simulink library "lib_Grid_DC_Dynamic"  (R2026a)
settings: Solver=VariableStepAuto
undefined symbols (not defined in the file): DC, From_nodes, Load_busesDC, op_Grid_DC_Dynamic, R_Loads_DC
settings Model: Creator=atomas  LastModifiedBy=atomas

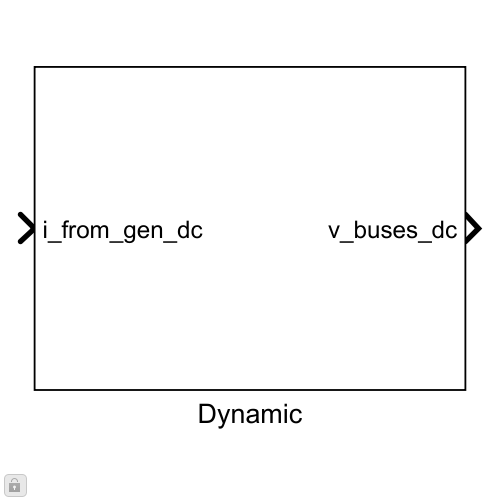
[thumbnail: Simulink's stored preview of the top-level diagram]
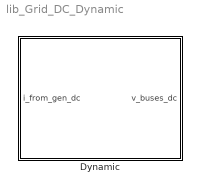
== system lib_Grid_DC_Dynamic ==
  Dynamic : Subsystem  VariantControl=Dynamic

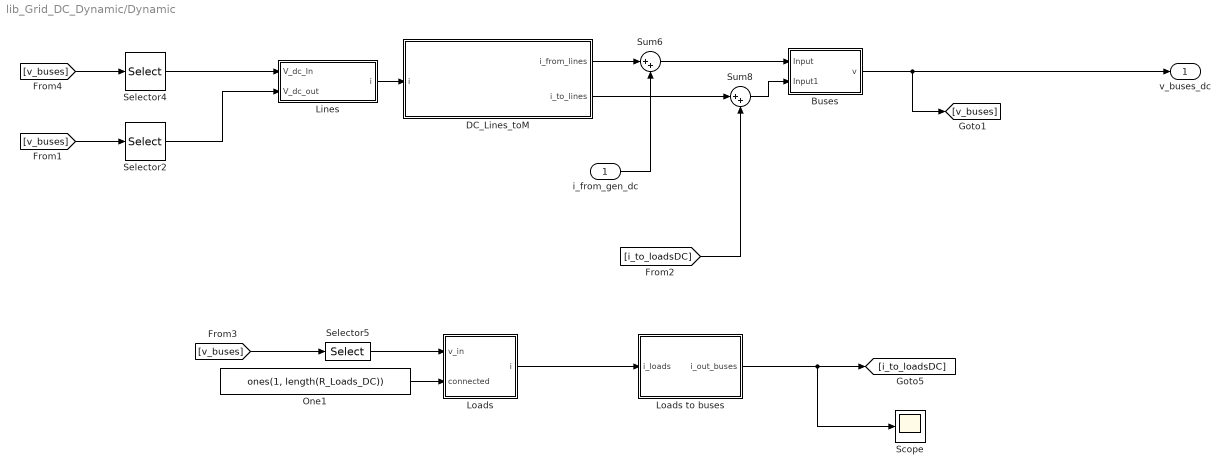
== system lib_Grid_DC_Dynamic/Dynamic ==
  i_from_gen_dc : Inport
  Buses : Subsystem
  DC_Lines_toM : Subsystem  TreatAsAtomicUnit=on
  Lines : Subsystem
  Loads : Subsystem
  Loads to buses : Subsystem
  One1 : Constant  Value=ones(1, length(R_Loads_DC))  VectorParams1D=off  OutDataTypeStr=Inherit: Inherit via back propagation
  Scope : Scope
      settings: ActiveDisplayYMinimum=-0.01246  ActiveDisplayYMaximum=0.11218
  Selector2 : Selector  NumberOfDimensions=2  InputPortWidth=Nnodes  IndexOptions=Select all,Index vector (dialog)  Indices=From_nodes,DC.to  OutputSizes=1,1
  Selector4 : Selector  NumberOfDimensions=2  InputPortWidth=Nnodes  IndexOptions=Select all,Index vector (dialog)  Indices=From_nodes,DC.from  OutputSizes=1,1
  Selector5 : Selector  NumberOfDimensions=2  InputPortWidth=Nnodes  IndexOptions=Select all,Index vector (dialog)  Indices=1,Load_busesDC  OutputSizes=1,1
  Sum6 : Sum  Inputs=|++
  Sum8 : Sum  Inputs=|++
  v_buses_dc : Outport
  wires:
  Buses/1(v) -> v_buses_dc/1, [v_buses]
  [v_buses] -> Selector2/1
  Selector2/1 -> Lines/2(V_dc_out)
  Sum6/1 -> Buses/1(Input)
  Selector4/1 -> Lines/1(V_dc_In)
  Loads/1(i) -> Loads to buses/1(i_loads)
  Selector5/1 -> Loads/1(v_in)
  i_from_gen_dc/1 -> Sum6/2
  Sum8/1 -> Buses/2(Input1)
  DC_Lines_toM/2(i_to_lines) -> Sum8/1
  DC_Lines_toM/1(i_from_lines) -> Sum6/1
  [v_buses] -> Selector4/1
  [i_to_loadsDC] -> Sum8/2
  Lines/1(i) -> DC_Lines_toM/1(i)
  One1/1 -> Loads/2(connected)
  Loads to buses/1(i_out_buses) -> Scope/1, [i_to_loadsDC]
  [v_buses] -> Selector5/1

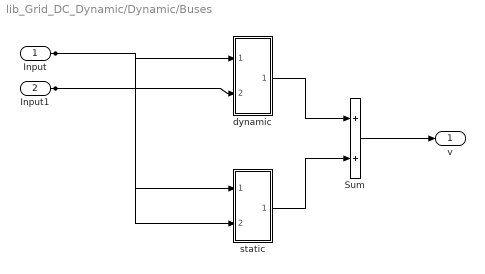
== system lib_Grid_DC_Dynamic/Dynamic/Buses ==
  Input : Inport
  Input1 : Inport  Port=2
  Sum : Sum
  dynamic : Subsystem  Variant=on
  static : Subsystem  Variant=on
  v : Outport
  wires:
  static/1(Out1) -> Sum/2
  Input1/1 -> static/2(In2), dynamic/2(In2)
  Input/1 -> static/1(In1), dynamic/1(In1)
  dynamic/1(Out1) -> Sum/1
  Sum/1 -> v/1

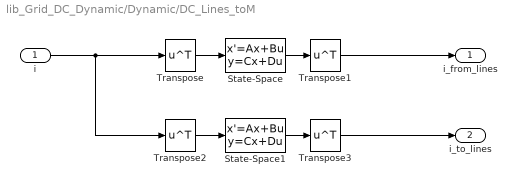
== system lib_Grid_DC_Dynamic/Dynamic/DC_Lines_toM ==
  i : Inport
  State-Space : StateSpace  A=[]  B=[]  C=[]  D=DC.Lines_toM  InitialCondition=0  ParameterTunability=Optimized
  State-Space1 : StateSpace  A=[]  B=[]  C=[]  D=DC.Lines_fromM  InitialCondition=0  ParameterTunability=Optimized
  Transpose{,1..3} (4 alike) : Math  Operator=transpose
  i_from_lines : Outport
  i_to_lines : Outport  Port=2
  wires:
  Transpose2/1 -> State-Space1/1
  i/1 -> Transpose2/1, Transpose/1
  Transpose3/1 -> i_to_lines/1
  Transpose/1 -> State-Space/1
  State-Space1/1 -> Transpose3/1
  State-Space/1 -> Transpose1/1
  Transpose1/1 -> i_from_lines/1

== system lib_Grid_DC_Dynamic/Dynamic/Lines ==
  V_dc_In : Inport
  V_dc_out : Inport  Port=2
  Dynamic : Subsystem  Variant=on
  Static : Subsystem  Variant=on
  Sum4 : Sum
  i : Outport
  wires:
  Static/1(Out1) -> Sum4/2
  V_dc_out/1 -> Static/2(In2), Dynamic/2(In2)
  V_dc_In/1 -> Static/1(In1), Dynamic/1(In1)
  Dynamic/1(Out1) -> Sum4/1
  Sum4/1 -> i/1

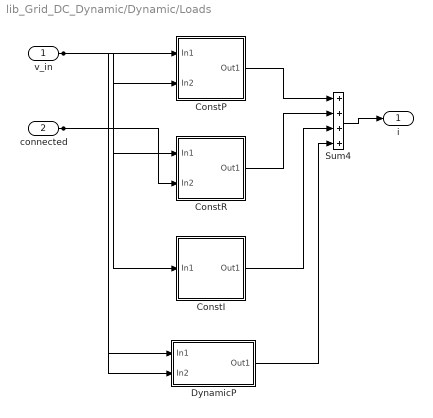
== system lib_Grid_DC_Dynamic/Dynamic/Loads ==
  v_in : Inport
  connected : Inport  Port=2
  ConstI : Subsystem  Variant=on
  ConstP : Subsystem  Variant=on
  ConstR : Subsystem  Variant=on
  DynamicP : Subsystem  Variant=on
  Sum4 : Sum  Inputs=++++
  i : Outport
  wires:
  DynamicP/1(Out1) -> Sum4/4
  connected/1 -> DynamicP/2(In2), ConstI/1(In1), ConstP/2(In2), ConstR/2(In2)
  v_in/1 -> DynamicP/1(In1), ConstP/1(In1), ConstR/1(In1)
  ConstI/1(Out1) -> Sum4/3
  ConstP/1(Out1) -> Sum4/1
  ConstR/1(Out1) -> Sum4/2
  Sum4/1 -> i/1

== system lib_Grid_DC_Dynamic/Dynamic/Loads to buses ==
  i_loads : Inport
  LoadsM : Subsystem  TreatAsAtomicUnit=on
  i_out_buses : Outport
  wires:
  i_loads/1 -> LoadsM/1(i)
  LoadsM/1(i_out_buses) -> i_out_buses/1

== system lib_Grid_DC_Dynamic/Dynamic/Buses/dynamic ==
  note: 1) Add Subsystem or Model blocks as valid variant choices.
      | 2) You cannot connect blocks at this level. At simulation, connectivity is automatically
      | determined, based on the active variant and port name matching.
  In1 : Inport
  In2 : Inport  Port=2
  Active : Subsystem  VariantControl=has_busDC_c1 == 1
  Bypass : Subsystem  VariantControl=(default)
  Out1 : Outport

== system lib_Grid_DC_Dynamic/Dynamic/Buses/static ==
  note: 1) Add Subsystem or Model blocks as valid variant choices.
      | 2) You cannot connect blocks at this level. At simulation, connectivity is automatically
      | determined, based on the active variant and port name matching.
  In1 : Inport
  In2 : Inport  Port=2
  Active : Subsystem  VariantControl=has_busDC_c2 == 1
  Bypass : Subsystem  VariantControl=(default)
  Out1 : Outport

== system lib_Grid_DC_Dynamic/Dynamic/Lines/Dynamic ==
  note: 1) Add Subsystem or Model blocks as valid variant choices.
      | 2) You cannot connect blocks at this level. At simulation, connectivity is automatically
      | determined, based on the active variant and port name matching.
  In1 : Inport
  In2 : Inport  Port=2
  Active : Subsystem  VariantControl=has_lineDC_c1 == 1
  Bypass : Subsystem  VariantControl=(default)
  Out1 : Outport

== system lib_Grid_DC_Dynamic/Dynamic/Lines/Static ==
  note: 1) Add Subsystem or Model blocks as valid variant choices.
      | 2) You cannot connect blocks at this level. At simulation, connectivity is automatically
      | determined, based on the active variant and port name matching.
  In1 : Inport
  In2 : Inport  Port=2
  Active : Subsystem  VariantControl=has_lineDC_c2 == 1
  Bypass : Subsystem  VariantControl=(default)
  Out1 : Outport

== system lib_Grid_DC_Dynamic/Dynamic/Loads/ConstI ==
  note: 1) Add Subsystem or Model blocks as valid variant choices.
      | 2) You cannot connect blocks at this level. At simulation, connectivity is automatically
      | determined, based on the active variant and port name matching.
  In1 : Inport
  Active : Subsystem  VariantControl=has_loadDC_c3 == 1
  Bypass : Subsystem  VariantControl=(default)
  Out1 : Outport

== system lib_Grid_DC_Dynamic/Dynamic/Loads/ConstP ==
  note: 1) Add Subsystem or Model blocks as valid variant choices.
      | 2) You cannot connect blocks at this level. At simulation, connectivity is automatically
      | determined, based on the active variant and port name matching.
  In1 : Inport
  In2 : Inport  Port=2
  Active : Subsystem  VariantControl=has_loadDC_c2 == 1
  Bypass : Subsystem  VariantControl=(default)
  Out1 : Outport

== system lib_Grid_DC_Dynamic/Dynamic/Loads/ConstR ==
  note: 1) Add Subsystem or Model blocks as valid variant choices.
      | 2) You cannot connect blocks at this level. At simulation, connectivity is automatically
      | determined, based on the active variant and port name matching.
  In1 : Inport
  In2 : Inport  Port=2
  Active : Subsystem  VariantControl=has_loadDC_c1 == 1
  Bypass : Subsystem  VariantControl=(default)
  Out1 : Outport

== system lib_Grid_DC_Dynamic/Dynamic/Loads/DynamicP ==
  note: 1) Add Subsystem or Model blocks as valid variant choices.
      | 2) You cannot connect blocks at this level. At simulation, connectivity is automatically
      | determined, based on the active variant and port name matching.
  In1 : Inport
  In2 : Inport  Port=2
  Active : Subsystem  VariantControl=has_loadDC_c4 == 1
  Bypass : Subsystem  VariantControl=(default)
  Out1 : Outport

== system lib_Grid_DC_Dynamic/Dynamic/Loads to buses/LoadsM ==
  i : Inport  Partition=on  PartitionDimension=1  PartitionWidth=1  PartitionOffset=0
  Assignment : Assignment  DiagnosticForDimensions=Warning  IndexOptions=Index vector (dialog)  Indices=Load_busesDC  OutputSizes=1
  For Each : ForEach  DisableCoverage=on
  Zero : Constant  Value=zeros(1,DC.Nbuses)  VectorParams1D=off  OutDataTypeStr=Inherit: Inherit via back propagation
  i_out_buses : Outport  ConcatenationDimension=1
  wires:
  Assignment/1 -> i_out_buses/1
  i/1 -> Assignment/2
  Zero/1 -> Assignment/1

== system lib_Grid_DC_Dynamic/Dynamic/Buses/dynamic/Active ==
  In1 : Inport
  In2 : Inport  Port=2
  Impl : Subsystem
  Out1 : Outport
  wires:
  Impl/1(v) -> Out1/1
  In2/1 -> Impl/2(i_out)
  In1/1 -> Impl/1(i_in)

== system lib_Grid_DC_Dynamic/Dynamic/Buses/dynamic/Bypass ==
  In1 : Inport
  In2 : Inport  Port=2
  Term1 : Terminator
  Term2 : Terminator
  Zero1 : Constant  Value=zeros(1, max(1, DC.Nbuses))  VectorParams1D=off
  Out1 : Outport
  wires:
  Zero1/1 -> Out1/1
  In2/1 -> Term2/1
  In1/1 -> Term1/1

== system lib_Grid_DC_Dynamic/Dynamic/Buses/static/Active ==
  In1 : Inport
  In2 : Inport  Port=2
  Impl : Subsystem
  Out1 : Outport
  wires:
  Impl/1(v) -> Out1/1
  In2/1 -> Impl/2(i_out)
  In1/1 -> Impl/1(i_in)

== system lib_Grid_DC_Dynamic/Dynamic/Buses/static/Bypass ==
  In1 : Inport
  In2 : Inport  Port=2
  Term1 : Terminator
  Term2 : Terminator
  Zero1 : Constant  Value=zeros(1, max(1, DC.Nbuses))  VectorParams1D=off
  Out1 : Outport
  wires:
  Zero1/1 -> Out1/1
  In2/1 -> Term2/1
  In1/1 -> Term1/1

== system lib_Grid_DC_Dynamic/Dynamic/Lines/Dynamic/Active ==
  In1 : Inport
  In2 : Inport  Port=2
  Impl : Subsystem
  Out1 : Outport
  wires:
  Impl/1(i) -> Out1/1
  In2/1 -> Impl/2(V_dc_Out)
  In1/1 -> Impl/1(V_dc_In)

== system lib_Grid_DC_Dynamic/Dynamic/Lines/Dynamic/Bypass ==
  In1 : Inport
  In2 : Inport  Port=2
  Term1 : Terminator
  Term2 : Terminator
  Zero1 : Constant  Value=zeros(1, max(1, length(DC.from)))  VectorParams1D=off
  Out1 : Outport
  wires:
  Zero1/1 -> Out1/1
  In2/1 -> Term2/1
  In1/1 -> Term1/1

== system lib_Grid_DC_Dynamic/Dynamic/Lines/Static/Active ==
  In1 : Inport
  In2 : Inport  Port=2
  Impl : Subsystem
  Out1 : Outport
  wires:
  Impl/1(i) -> Out1/1
  In2/1 -> Impl/2(V_dc_Out)
  In1/1 -> Impl/1(V_dc_In)

== system lib_Grid_DC_Dynamic/Dynamic/Lines/Static/Bypass ==
  In1 : Inport
  In2 : Inport  Port=2
  Term1 : Terminator
  Term2 : Terminator
  Zero1 : Constant  Value=zeros(1, max(1, length(DC.from)))  VectorParams1D=off
  Out1 : Outport
  wires:
  Zero1/1 -> Out1/1
  In2/1 -> Term2/1
  In1/1 -> Term1/1

== system lib_Grid_DC_Dynamic/Dynamic/Loads/ConstI/Active ==
  In1 : Inport
  Impl : Subsystem
  Out1 : Outport
  wires:
  Impl/1(i) -> Out1/1
  In1/1 -> Impl/1(connected)

== system lib_Grid_DC_Dynamic/Dynamic/Loads/ConstI/Bypass ==
  In1 : Inport
  Term1 : Terminator
  Zero1 : Constant  Value=zeros(1, max(1, length(R_Loads_DC)))  VectorParams1D=off
  Out1 : Outport
  wires:
  Zero1/1 -> Out1/1
  In1/1 -> Term1/1

== system lib_Grid_DC_Dynamic/Dynamic/Loads/ConstP/Active ==
  In1 : Inport
  In2 : Inport  Port=2
  Impl : Subsystem
  Out1 : Outport
  wires:
  Impl/1(i) -> Out1/1
  In2/1 -> Impl/2(connected)
  In1/1 -> Impl/1(v_in)

== system lib_Grid_DC_Dynamic/Dynamic/Loads/ConstP/Bypass ==
  In1 : Inport
  In2 : Inport  Port=2
  Term1 : Terminator
  Term2 : Terminator
  Zero1 : Constant  Value=zeros(1, max(1, length(R_Loads_DC)))  VectorParams1D=off
  Out1 : Outport
  wires:
  Zero1/1 -> Out1/1
  In2/1 -> Term2/1
  In1/1 -> Term1/1

== system lib_Grid_DC_Dynamic/Dynamic/Loads/ConstR/Active ==
  In1 : Inport
  In2 : Inport  Port=2
  Impl : Subsystem
  Out1 : Outport
  wires:
  Impl/1(i) -> Out1/1
  In2/1 -> Impl/2(connected)
  In1/1 -> Impl/1(v_in)

== system lib_Grid_DC_Dynamic/Dynamic/Loads/ConstR/Bypass ==
  In1 : Inport
  In2 : Inport  Port=2
  Term1 : Terminator
  Term2 : Terminator
  Zero1 : Constant  Value=zeros(1, max(1, length(R_Loads_DC)))  VectorParams1D=off
  Out1 : Outport
  wires:
  Zero1/1 -> Out1/1
  In2/1 -> Term2/1
  In1/1 -> Term1/1

== system lib_Grid_DC_Dynamic/Dynamic/Loads/DynamicP/Active ==
  In1 : Inport
  In2 : Inport  Port=2
  Impl : Subsystem
  Out1 : Outport
  wires:
  Impl/1(i) -> Out1/1
  In2/1 -> Impl/2(connected)
  In1/1 -> Impl/1(v_in)

== system lib_Grid_DC_Dynamic/Dynamic/Loads/DynamicP/Bypass ==
  In1 : Inport
  In2 : Inport  Port=2
  Term1 : Terminator
  Term2 : Terminator
  Zero1 : Constant  Value=zeros(1, max(1, length(R_Loads_DC)))  VectorParams1D=off
  Out1 : Outport
  wires:
  Zero1/1 -> Out1/1
  In2/1 -> Term2/1
  In1/1 -> Term1/1

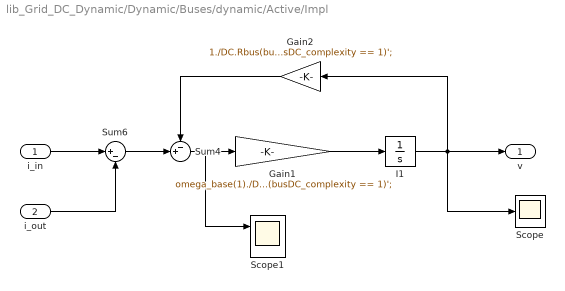
== system lib_Grid_DC_Dynamic/Dynamic/Buses/dynamic/Active/Impl ==
  i_in : Inport
  i_out : Inport  Port=2
  Gain1 : Gain  Gain=omega_base(1)./DC.CbusDC(busDC_complexity == 1)';
  Gain2 : Gain  Gain=1./DC.Rbus(busDC_complexity == 1)';
  I1 : Integrator  InitialCondition=op_Grid_DC_Dynamic.Buses_dynamic_Active_Impl_I1
  Scope : Scope
      settings: ActiveDisplayYMinimum=0.9  ActiveDisplayYMaximum=1.1
  Scope1 : Scope  NumInputPorts=2
      settings: ActiveDisplayYMinimum=-0.35489510103335586  ActiveDisplayYMaximum=0.27003394850354928  DataLoggingVariableName=ScopeData5
  Sum4 : Sum  Inputs=-+|
  Sum6 : Sum  Inputs=|+-
  v : Outport
  wires:
  Gain1/1 -> I1/1
  i_out/1 -> Sum6/2
  Sum6/1 -> Sum4/2
  Sum4/1 -> Gain1/1, Scope1/1
  i_in/1 -> Sum6/1
  I1/1 -> Gain2/1, v/1, Scope/1
  Gain2/1 -> Sum4/1

== system lib_Grid_DC_Dynamic/Dynamic/Buses/static/Active/Impl ==
  i_in : Inport
  i_out : Inport  Port=2
  Gain : Gain  Gain=1/1e-6
  LPF_d1 : Subsystem
  Sum1 : Sum  Inputs=+-
  v : Outport
  wires:
  LPF_d1/1(v_buses_dc) -> v/1
  Gain/1 -> LPF_d1/1(In1)
  i_out/1 -> Sum1/2
  i_in/1 -> Sum1/1
  Sum1/1 -> Gain/1

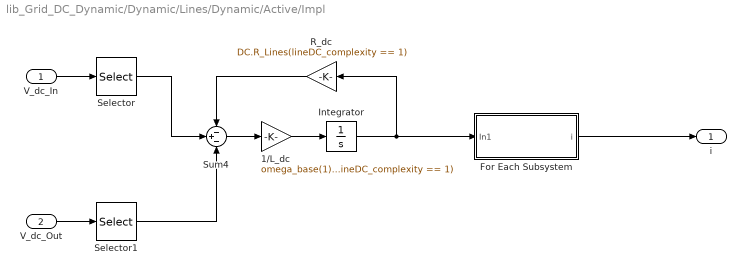
== system lib_Grid_DC_Dynamic/Dynamic/Lines/Dynamic/Active/Impl ==
  V_dc_In : Inport
  V_dc_Out : Inport  Port=2
  1/L_dc : Gain  Gain=omega_base(1)./DC.L_Lines(lineDC_complexity == 1)
  For Each Subsystem : Subsystem  TreatAsAtomicUnit=on
  Integrator : Integrator  InitialCondition=op_Grid_DC_Dynamic.Lines_Dynamic_Active_Impl_Integrator
  R_dc : Gain  Gain=DC.R_Lines(lineDC_complexity == 1)
  Selector : Selector  NumberOfDimensions=2  InputPortWidth=3  IndexOptions=Index vector (dialog),Index vector (dialog)  Indices=1,find(lineDC_complexity == 1)  OutputSizes=1,1
  Selector1 : Selector  NumberOfDimensions=2  InputPortWidth=3  IndexOptions=Index vector (dialog),Index vector (dialog)  Indices=1,find(lineDC_complexity == 1)  OutputSizes=1,1
  Sum4 : Sum  Inputs=-+-
  i : Outport
  wires:
  Selector1/1 -> Sum4/3
  Selector/1 -> Sum4/2
  V_dc_In/1 -> Selector/1
  V_dc_Out/1 -> Selector1/1
  For Each Subsystem/1(i) -> i/1
  R_dc/1 -> Sum4/1
  1/L_dc/1 -> Integrator/1
  Sum4/1 -> 1/L_dc/1
  Integrator/1 -> R_dc/1, For Each Subsystem/1(In1)

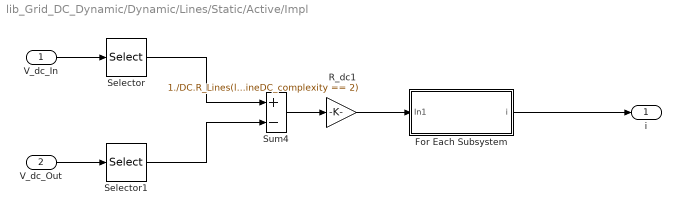
== system lib_Grid_DC_Dynamic/Dynamic/Lines/Static/Active/Impl ==
  V_dc_In : Inport
  V_dc_Out : Inport  Port=2
  For Each Subsystem : Subsystem  TreatAsAtomicUnit=on
  R_dc1 : Gain  Gain=1./DC.R_Lines(lineDC_complexity == 2)
  Selector : Selector  NumberOfDimensions=2  InputPortWidth=3  IndexOptions=Index vector (dialog),Index vector (dialog)  Indices=1,find(lineDC_complexity == 2)  OutputSizes=1,1
  Selector1 : Selector  NumberOfDimensions=2  InputPortWidth=3  IndexOptions=Index vector (dialog),Index vector (dialog)  Indices=1,find(lineDC_complexity == 2)  OutputSizes=1,1
  Sum4 : Sum  Inputs=+-
  i : Outport
  wires:
  Selector1/1 -> Sum4/2
  V_dc_Out/1 -> Selector1/1
  Selector/1 -> Sum4/1
  V_dc_In/1 -> Selector/1
  For Each Subsystem/1(i) -> i/1
  R_dc1/1 -> For Each Subsystem/1(In1)
  Sum4/1 -> R_dc1/1

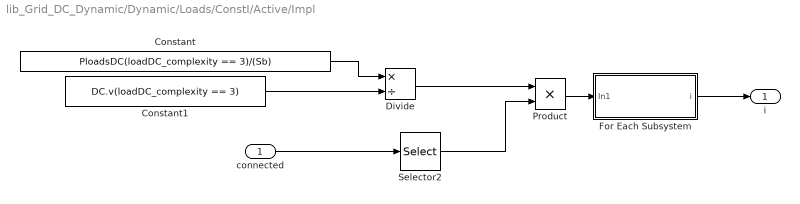
== system lib_Grid_DC_Dynamic/Dynamic/Loads/ConstI/Active/Impl ==
  connected : Inport
  Constant : Constant  Value=PloadsDC(loadDC_complexity == 3)/(Sb)
  Constant1 : Constant  Value=DC.v(loadDC_complexity == 3)
  Divide : Product  Inputs=*/
  For Each Subsystem : Subsystem  TreatAsAtomicUnit=on
  Product : Product
  Selector2 : Selector  InputPortWidth=length(R_Loads_DC)  IndexOptions=Index vector (dialog)  Indices=find(loadDC_complexity == 3)  OutputSizes=1
  i : Outport
  wires:
  Divide/1 -> Product/1
  Constant1/1 -> Divide/2
  Constant/1 -> Divide/1
  For Each Subsystem/1(i) -> i/1
  Product/1 -> For Each Subsystem/1(In1)
  Selector2/1 -> Product/2
  connected/1 -> Selector2/1

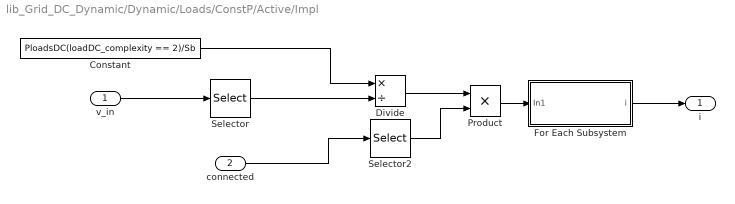
== system lib_Grid_DC_Dynamic/Dynamic/Loads/ConstP/Active/Impl ==
  v_in : Inport
  connected : Inport  Port=2
  Constant : Constant  Value=PloadsDC(loadDC_complexity == 2)/Sb  VectorParams1D=off
  Divide : Product  Inputs=*/
  For Each Subsystem : Subsystem  TreatAsAtomicUnit=on
  Product : Product
  Selector : Selector  NumberOfDimensions=2  InputPortWidth=3  IndexOptions=Index vector (dialog),Index vector (dialog)  Indices=1,find(loadDC_complexity == 2)  OutputSizes=1,1
  Selector2 : Selector  InputPortWidth=length(R_Loads_DC)  IndexOptions=Index vector (dialog)  Indices=find(loadDC_complexity == 2)  OutputSizes=1
  i : Outport
  wires:
  For Each Subsystem/1(i) -> i/1
  Product/1 -> For Each Subsystem/1(In1)
  Selector/1 -> Divide/2
  v_in/1 -> Selector/1
  Selector2/1 -> Product/2
  connected/1 -> Selector2/1
  Divide/1 -> Product/1
  Constant/1 -> Divide/1

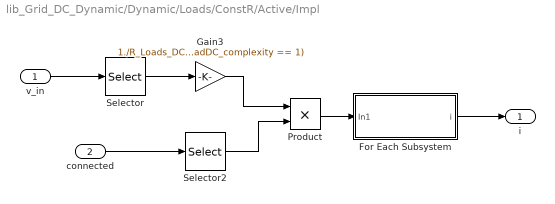
== system lib_Grid_DC_Dynamic/Dynamic/Loads/ConstR/Active/Impl ==
  v_in : Inport
  connected : Inport  Port=2
  For Each Subsystem : Subsystem  TreatAsAtomicUnit=on
  Gain3 : Gain  Gain=1./R_Loads_DC(loadDC_complexity == 1)
  Product : Product
  Selector : Selector  NumberOfDimensions=2  InputPortWidth=3  IndexOptions=Index vector (dialog),Index vector (dialog)  Indices=1,find(loadDC_complexity == 1)  OutputSizes=1,1
  Selector2 : Selector  InputPortWidth=length(R_Loads_DC)  IndexOptions=Index vector (dialog)  Indices=find(loadDC_complexity == 1)  OutputSizes=1
  i : Outport
  wires:
  For Each Subsystem/1(i) -> i/1
  Product/1 -> For Each Subsystem/1(In1)
  Selector/1 -> Gain3/1
  v_in/1 -> Selector/1
  Selector2/1 -> Product/2
  connected/1 -> Selector2/1
  Gain3/1 -> Product/1

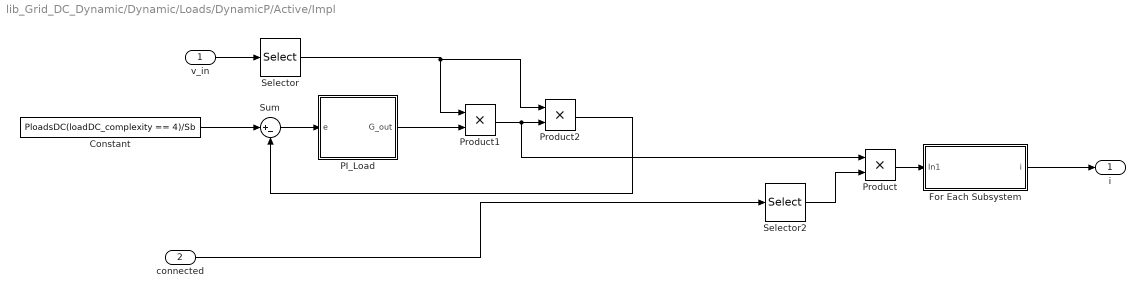
== system lib_Grid_DC_Dynamic/Dynamic/Loads/DynamicP/Active/Impl ==
  v_in : Inport
  connected : Inport  Port=2
  Constant : Constant  Value=PloadsDC(loadDC_complexity == 4)/Sb
  For Each Subsystem : Subsystem  TreatAsAtomicUnit=on
  PI_Load : Subsystem
  Product : Product
  Product1 : Product
  Product2 : Product
  Selector : Selector  NumberOfDimensions=2  InputPortWidth=3  IndexOptions=Index vector (dialog),Index vector (dialog)  Indices=1,find(loadDC_complexity == 4)  OutputSizes=1,1
  Selector2 : Selector  InputPortWidth=length(R_Loads_DC)  IndexOptions=Index vector (dialog)  Indices=find(loadDC_complexity == 4)  OutputSizes=1
  Sum : Sum  Inputs=|+-
  i : Outport
  wires:
  Sum/1 -> PI_Load/1(e)
  PI_Load/1(G_out) -> Product1/2
  Product/1 -> For Each Subsystem/1(In1)
  For Each Subsystem/1(i) -> i/1
  Product1/1 -> Product2/2, Product/1
  Product2/1 -> Sum/2
  connected/1 -> Selector2/1
  Constant/1 -> Sum/1
  Selector2/1 -> Product/2
  v_in/1 -> Selector/1
  Selector/1 -> Product1/1, Product2/1

== system lib_Grid_DC_Dynamic/Dynamic/Buses/static/Active/Impl/LPF_d1 ==
  In1 : Inport
  Gain : Gain  Gain=100
  I : Integrator  InitialCondition=op_Grid_DC_Dynamic.Buses_static_Active_Impl_LPF_d1_I
  Sum4 : Sum  Inputs=|+-
  v_buses_dc : Outport
  wires:
  I/1 -> Sum4/2, v_buses_dc/1
  In1/1 -> Sum4/1
  Sum4/1 -> Gain/1
  Gain/1 -> I/1

== system lib_Grid_DC_Dynamic/Dynamic/Lines/Dynamic/Active/Impl/For Each Subsystem ==
  In1 : Inport  Partition=on  PartitionDimension=1  PartitionWidth=1  PartitionOffset=0
  Assignment : Assignment  DiagnosticForDimensions=Warning  IndexOptions=Index vector (dialog)  Indices=find(lineDC_complexity == 1)  OutputSizes=1
  For Each : ForEach  DisableCoverage=on
  Zero : Constant  Value=zeros(1,length(DC.from))  VectorParams1D=off  OutDataTypeStr=Inherit: Inherit via back propagation
  i : Outport  ConcatenationDimension=1
  wires:
  Zero/1 -> Assignment/1
  Assignment/1 -> i/1
  In1/1 -> Assignment/2

== system lib_Grid_DC_Dynamic/Dynamic/Lines/Static/Active/Impl/For Each Subsystem ==
  In1 : Inport  Partition=on  PartitionDimension=1  PartitionWidth=1  PartitionOffset=0
  Assignment : Assignment  DiagnosticForDimensions=Warning  IndexOptions=Index vector (dialog)  Indices=find(lineDC_complexity == 2)  OutputSizes=1
  For Each : ForEach  DisableCoverage=on
  Zero : Constant  Value=zeros(1,length(DC.from))  VectorParams1D=off  OutDataTypeStr=Inherit: Inherit via back propagation
  i : Outport  ConcatenationDimension=1
  wires:
  Zero/1 -> Assignment/1
  Assignment/1 -> i/1
  In1/1 -> Assignment/2

== system lib_Grid_DC_Dynamic/Dynamic/Loads/ConstI/Active/Impl/For Each Subsystem ==
  In1 : Inport  Partition=on  PartitionDimension=1  PartitionWidth=1  PartitionOffset=0
  Assignment : Assignment  DiagnosticForDimensions=Warning  IndexOptions=Index vector (dialog)  Indices=find(loadDC_complexity == 3)  OutputSizes=1
  For Each : ForEach  DisableCoverage=on
  Zero : Constant  Value=zeros(1,length(R_Loads_DC))  VectorParams1D=off  OutDataTypeStr=Inherit: Inherit via back propagation
  i : Outport  ConcatenationDimension=1
  wires:
  Zero/1 -> Assignment/1
  Assignment/1 -> i/1
  In1/1 -> Assignment/2

== system lib_Grid_DC_Dynamic/Dynamic/Loads/ConstP/Active/Impl/For Each Subsystem ==
  In1 : Inport  Partition=on  PartitionDimension=1  PartitionWidth=1  PartitionOffset=0
  Assignment : Assignment  DiagnosticForDimensions=Warning  IndexOptions=Index vector (dialog)  Indices=find(loadDC_complexity == 2)  OutputSizes=1
  For Each : ForEach  DisableCoverage=on
  Zero : Constant  Value=zeros(1,length(R_Loads_DC))  VectorParams1D=off  OutDataTypeStr=Inherit: Inherit via back propagation
  i : Outport  ConcatenationDimension=1
  wires:
  Zero/1 -> Assignment/1
  Assignment/1 -> i/1
  In1/1 -> Assignment/2

== system lib_Grid_DC_Dynamic/Dynamic/Loads/ConstR/Active/Impl/For Each Subsystem ==
  In1 : Inport  Partition=on  PartitionDimension=1  PartitionWidth=1  PartitionOffset=0
  Assignment : Assignment  DiagnosticForDimensions=Warning  IndexOptions=Index vector (dialog)  Indices=find(loadDC_complexity == 1)  OutputSizes=1
  For Each : ForEach  DisableCoverage=on
  Zero : Constant  Value=zeros(1,length(R_Loads_DC))  VectorParams1D=off  OutDataTypeStr=Inherit: Inherit via back propagation
  i : Outport  ConcatenationDimension=1
  wires:
  Zero/1 -> Assignment/1
  Assignment/1 -> i/1
  In1/1 -> Assignment/2

== system lib_Grid_DC_Dynamic/Dynamic/Loads/DynamicP/Active/Impl/For Each Subsystem ==
  In1 : Inport  Partition=on  PartitionDimension=1  PartitionWidth=1  PartitionOffset=0
  Assignment : Assignment  DiagnosticForDimensions=Warning  IndexOptions=Index vector (dialog)  Indices=find(loadDC_complexity == 4)  OutputSizes=1
  For Each : ForEach  DisableCoverage=on
  Zero : Constant  Value=zeros(1,length(R_Loads_DC))  VectorParams1D=off  OutDataTypeStr=Inherit: Inherit via back propagation
  i : Outport  ConcatenationDimension=1
  wires:
  Zero/1 -> Assignment/1
  Assignment/1 -> i/1
  In1/1 -> Assignment/2

== system lib_Grid_DC_Dynamic/Dynamic/Loads/DynamicP/Active/Impl/PI_Load ==
  e : Inport
  Gain : Gain  Gain=0.1/(100*pi)
  Gain1 : Gain  Gain=0.2/(100*pi)
  I : Integrator  InitialCondition=op_Grid_DC_Dynamic.Loads_DynamicP_Active_Impl_PI_Load_I
  Sum10 : Sum  Inputs=|++
  G_out : Outport
  wires:
  Sum10/1 -> G_out/1
  Gain/1 -> Sum10/1
  I/1 -> Sum10/2
  Gain1/1 -> I/1
  e/1 -> Gain/1, Gain1/1
